simulink model "hopper_6dof"  (R2026b)
settings: Solver=FixedStepAuto  StopTime=tgrid(end)  FixedStep=1e-3  RelTol=1e-5
undefined symbols (not defined in the file): cg_init, controller_start_time, fdir_params, fsw_latency, fsw_period, g, IN, K1flat, K1flat_lo, K2grid, Klqi, nav_dt, nav_g, nav_init, nav_Qc, nav_reset, OUT, p, sensor_params, Target_Trajectory, tgrid, u_hold_command, unom, VEH
libraries: fl_lib x43, nesl_utility x31, SimscapeFluids_lib x13, slpidlib x3, simulink_extras x2, commrandsrc3 x1, dspsrcs4 x1, matrix_library x1, aerolibutil x1
(part 4 of 6)

== system hopper_6dof/Mass_Propulsion/Propulsion/Propulsion_Fluid_Network/Fluid_Network/FBB ==
  Acuation Delay : TransportDelay  DelayTime=0.075  InitialOutput=1  BufferSize=28672
  Constant5 : Constant  Value=0
  Constant6 : Constant
  F Orifice : SimscapeFluids_lib/Gas/Valves & Orifices/Orifice (G)  orifice_type=foundation.enum.constant_variable.constant  orifice_parameterization=fluids.gas.valves_orifices.enum.OrificeParameterization.Area  opening_characteristic=fluids.gas.valves_orifices.enum.OpeningCharacteristics.Linear  Cv_constant=4  Cv_max=4  L_Cv_TLU=0 : 0.2 : 1  Cv_TLU=[1e-06, .8, 1.6, 2.4, 3.2, 4]  xT_Cv=0.7  Kv_constant=3.6  Kv_max=3.6  L_Kv_TLU=0 : 0.2 : 1  Kv_TLU=[1e-06, .72, 1.44, 2.16, 2.88, 3.6]  xT_Kv=0.7  C_constant=12 l/(bar*s)  B_crit_constant=0.3  C_max=12 l/(bar*s)  B_crit_linear=0.3  L_C_TLU=0 : 0.2 : 1  C_TLU=[1e-05, 2.4, 4.8, 7.2, 9.6, 12] l/(bar*s)  B_crit_TLU=0.3 * ones(1, 6)  m=0.5  T_ref_C=293.15 K  rho_ref_C=1.185 kg/m^3  orifice_area_constant=0.025477 in^2  orifice_area_max=1e-4 m^2  L_orifice_area_TLU=0 : 0.2 : 1  orifice_area_TLU=[1e-10, 2e-05, 4e-05, 6e-05, 8e-05, .0001] m^2  Cd=1  leakage_fraction=1e-6  smoothing_factor=0.01  B_lam=0.999  area=0.01 m^2
  FBang : SimscapeFluids_lib/Gas/Valves & Orifices/Flow Control Valves/Poppet Valve (G)  valve_seat_geometry=fluids.gas.valves_orifices.flow_control_valves.enum.ValveSeatGeometry.Sharp  cone_angle=120 deg  diam_ball=0.7 in  diam_orifice=0.05351 in  valve_parameterization=fluids.gas.valves_orifices.flow_control_valves.enum.OrificeParameterization.Geometry  Cd=1  Cv_max=4  xT_Cv=0.7  Kv_max=3.6  xT_Kv=0.7  C_max=12 l/(bar*s)  B_crit_linear=0.3  m=0.5  T_ref_C=293.15 K  rho_ref_C=1.185 kg/m^3  leakage_fraction=10^-9  smoothing_factor=0.01  B_lam=0.999  area=0.78 in^2  x0=0
  FTPT : Scope  Commented=on
      settings: ActiveDisplayYMinimum=469.21439817536259  ActiveDisplayYMaximum=560.55853932482523  DataLoggingVariableName=ScopeData5
  Mass & Energy Flow Rate Sensor (G)1 : fl_lib/Gas/Sensors/Flow Rate Sensor (G)  mass_flow_measure=true  volumetric_flow_measure=false  volumetric_flow_conditions=foundation.enum.volumetric_flow_conditions.actual  p_std=0.101325 MPa  T_std=20 degC  energy_flow_measure=true
  PS-Simulink Converter8 : nesl_utility/PS-Simulink Converter  PhysicalDomain=network_engine_domain  SubClassName=ps_output  LeftPortType=input  RightPortType=output  PseudoPeriodic=off  Frequencies=[]  VectorFormat=inherit  Unit=inherit  AffineConversion=off
  Pipe (G) : fl_lib/Gas/Elements/Pipe (G)  length=0.5 ft  area=0.049 in^2  Dh=0.25 in  length_add=0.1 m  roughness=0.0015 mm  Re_lam=2000  Re_tur=4000  shape_factor=64  Nu_lam=3.66  dynamic_compressibility=true  inertia=false  p_init=4500 psi  p_init_priority=foundation.enum.Priority.High  T_init=293.15 K  T_init_priority=foundation.enum.Priority.High  mdot_init=0 kg/s  mdot_init_priority=foundation.enum.Priority.High  p_nominal=0.101325 MPa  T_nominal=293.15 K
  Pressurant Mass Flow Rate FSide : Scope  Commented=on
      settings: ActiveDisplayYMinimum=-1  ActiveDisplayYMaximum=1  DataLoggingVariableName=ScopeData15
  Rate Limiter1 : RateLimiter  RisingSlewLimit=100  FallingSlewLimit=-100  SampleTimeMode=inherited
  Simulink-PS Converter4 : nesl_utility/Simulink-PS Converter  PhysicalDomain=network_engine_domain  SubClassName=ps_input  LeftPortType=input  RightPortType=output  PseudoPeriodic=off  Frequencies=[]  NoiseDistribution=none  NoiseParameters=[]  Unit=1  AffineConversion=off  FilteringAndDerivatives=filter  SimscapeFilterOrder=1  InputFilterTimeConstant=0.001  UdotUserProvided=0
  Subsystem Reference : Subsystem  ReferencedSubsystem=PT  max_press=5000  lower_val=4  upper_val=20
  Switch1 : Switch  Criteria=u2 > Threshold  Threshold=500  SaturateOnIntegerOverflow=off  InputSameDT=off
  Valve State3 : Scope  Commented=on
      settings: ActiveDisplayYMinimum=-1  ActiveDisplayYMaximum=1  DataLoggingVariableName=ScopeData16
  Conn2 : PMIOPort  Side=Right
  Conn3 : PMIOPort  Port=2  Side=Left
  wires:
  Acuation Delay/1 -> Rate Limiter1/1
  Rate Limiter1/1 -> Valve State3/1, Simulink-PS Converter4/1
  Constant5/1 -> Switch1/1
  PS-Simulink Converter8/1 -> Pressurant Mass Flow Rate FSide/1
  Switch1/1 -> Acuation Delay/1
  Constant6/1 -> Switch1/3
  Subsystem Reference/1 -> FTPT/1, Switch1/2
  connections:
  Pipe (G)/RConn1 -- FBang/LConn1
  Conn3/RConn1 -- Pipe (G)/LConn1
  Mass & Energy Flow Rate Sensor (G)1/RConn1 -- Conn2/RConn1
  F Orifice/LConn1 -- FBang/RConn1
  FBang/LConn2 -- Simulink-PS Converter4/RConn1
  Subsystem Reference/LConn1 -- Mass & Energy Flow Rate Sensor (G)1/LConn1 -- F Orifice/RConn1
  PS-Simulink Converter8/LConn1 -- Mass & Energy Flow Rate Sensor (G)1/RConn2

== system hopper_6dof/Mass_Propulsion/Propulsion/Propulsion_Fluid_Network/Fluid_Network/Fuel Tank ==
  Fuel CdA : SimscapeFluids_lib/Thermal Liquid/Valves & Orifices/Orifice (TL)  Commented=on  orifice_type=foundation.enum.constant_variable.constant  constant_orifice_spec=fluids.thermal_liquid.valves.enum.ConstantOrificeSpec.Area  variable_orifice_spec=fluids.thermal_liquid.valves.enum.orifice_spec.linear  orifice_area_constant=100 mm^2  p_diff_TLU_constant=[-4, -3, -2, -1, -.5, 0, .5, 1, 2, 3, 4] MPa  vol_flow_TLU_constant=[-2.44, -2.12, -1.68, -1.22, -.84, 0, .85, 1.21, 1.7, 2.09, 2.41] .* 1e-3 m^3/s  mdot_TLU_constant=[-2.44, -2.12, -1.68, -1.22, -.84, 0, .85, 1.21, 1.7, 2.09, 2.41] kg/s  S_min=0 m  del_S=5e-3 m  open_orientation=fluids.thermal_liquid.valves.enum.orifice_orientation.positive  area_max=1e-4 m^2  area_leak=1e-10 m^2  S_TLU=[0, .002, .004, .007, .017] m  orifice_area_TLU=[1e-09, 2.0352e-07, 4.0736e-05, .00011438, .00034356] m^2  Cd=1  Re_c=150  smoothing_factor=0.01  pressure_recovery=simscape.enum.onoff.off  S_flow_TLU=[0, .002, .004, .007, .017] m  p_diff_TLU=[.3, .5, .7] MPa  vol_flow_TLU=1e-3 * [1.7e-05, 2e-05, 2.6e-05; .0035, .0045, .0053; .7, .9, 1.06; 1.96, 2.5, 3; 6, 7.7, 9.13] m^3/s  mdot_TLU=[1.7e-05, 2e-05, 2.6e-05; .0035, .0045, .0053; .7, .9, 1.06; 1.96, 2.5, 3; 6, 7.7, 9.13] kg/s  T_ref_in=293.15 K  p_ref_in=0.101325 MPa  area=0.01 m^2
  Fuel CdA1 : SimscapeFluids_lib/Thermal Liquid/Valves & Orifices/Orifice (TL)  orifice_type=foundation.enum.constant_variable.constant  constant_orifice_spec=fluids.thermal_liquid.valves.enum.ConstantOrificeSpec.Area  variable_orifice_spec=fluids.thermal_liquid.valves.enum.orifice_spec.linear  orifice_area_constant=100 mm^2  p_diff_TLU_constant=[-4, -3, -2, -1, -.5, 0, .5, 1, 2, 3, 4] MPa  vol_flow_TLU_constant=[-2.44, -2.12, -1.68, -1.22, -.84, 0, .85, 1.21, 1.7, 2.09, 2.41] .* 1e-3 m^3/s  mdot_TLU_constant=[-2.44, -2.12, -1.68, -1.22, -.84, 0, .85, 1.21, 1.7, 2.09, 2.41] kg/s  S_min=0 m  del_S=5e-3 m  open_orientation=fluids.thermal_liquid.valves.enum.orifice_orientation.positive  area_max=1e-4 m^2  area_leak=1e-10 m^2  S_TLU=[0, .002, .004, .007, .017] m  orifice_area_TLU=[1e-09, 2.0352e-07, 4.0736e-05, .00011438, .00034356] m^2  Cd=1  Re_c=150  smoothing_factor=0.01  pressure_recovery=simscape.enum.onoff.off  S_flow_TLU=[0, .002, .004, .007, .017] m  p_diff_TLU=[.3, .5, .7] MPa  vol_flow_TLU=1e-3 * [1.7e-05, 2e-05, 2.6e-05; .0035, .0045, .0053; .7, .9, 1.06; 1.96, 2.5, 3; 6, 7.7, 9.13] m^3/s  mdot_TLU=[1.7e-05, 2e-05, 2.6e-05; .0035, .0045, .0053; .7, .9, 1.06; 1.96, 2.5, 3; 6, 7.7, 9.13] kg/s  T_ref_in=293.15 K  p_ref_in=0.101325 MPa  area=0.01 m^2
  Fuel Liquid Level : Scope  Commented=on
      settings: ActiveDisplayYMinimum=-0.022349805039863307  ActiveDisplayYMaximum=0.600478334821636  DataLoggingVariableName=ScopeData6
  Fuel Mass Flow Rate : Scope  Commented=on
      settings: ActiveDisplayYMinimum=-0.023909818576535891  ActiveDisplayYMaximum=0.21591293735607325  DataLoggingVariableName=ScopeData7
  Fuel Mass Rate : Scope  Commented=on
      settings: ActiveDisplayYMinimum=-7.0412281631605644  ActiveDisplayYMaximum=46.559064275310185  DataLoggingVariableName=ScopeData18
  Fuel Tank (Jet A) : SimscapeFluids_lib/Thermal Liquid/Tanks & Accumulators/Tank (G-TL)  num_inlet=1  volume_total=30 l  volume_spec=fluids.thermal_liquid.tanks_accumulators.enum.TankVolumeSpec.Constant  tank_area=0.35 ft^2  level_TLU=[0, 3, 5] m  volume_TLU=[0, 4, 6] m^3  inlet_areas_A1B1=[1, 1] in^2  inlet_height_A2=0 m  inlet_area_A2=0.78 in^2  inlet_heights_A2B2=[.1, .1] m  inlet_areas_A2B2=[.01, .01] m^2  inlet_heights_A2B2C2=[.1, .1, .1] m  inlet_areas_A2B2C2=[.01, .01, .01] m^2  inlet_heights_A2B2C2D2=0.1 * ones(1, 4) m  inlet_areas_A2B2C2D2=0.01 * ones(1, 4) m^2  inlet_heights_A2B2C2D2E2=0.1 * ones(1, 5) m  inlet_areas_A2B2C2D2E2=0.01 * ones(1, 5) m^2  inlet_heights_A2B2C2D2E2F2=0.1 * ones(1, 6) m  inlet_areas_A2B2C2D2E2F2=0.01 * ones(1, 6) m^2  capacity_check=0  max_liquid_capacity=55 l  g=9.81 m/s^2  level_specify=off  level_priority=None  level=19 in  level_nominal_specify=off  level_nominal_value=1  level_nominal_unit=m  volume_liquid_specify=off  volume_liquid_priority=None  volume_liquid=15.18 l  volume_liquid_nominal_specify=off  volume_liquid_nominal_value=1  volume_liquid_nominal_unit=m^3  mass_liquid_specify=on  mass_liquid_priority=High  mass_liquid=20 kg  mass_liquid_nominal_specify=off  mass_liquid_nominal_value=1  mass_liquid_nominal_unit=kg  T_liquid_specify=off  T_liquid_priority=High  T_liquid=293.15 K  T_liquid_nominal_specify=off  T_liquid_nominal_value=1  T_liquid_nominal_unit=K  p_gas_specify=on  p_gas_priority=High  p_gas=500 psi  p_gas_nominal_specify=off  p_gas_nominal_value=1  p_gas_nominal_unit=MPa  T_gas_specify=off  T_gas_priority=High  T_gas=293.15 K  T_gas_nominal_specify=off  T_gas_nominal_value=1  T_gas_nominal_unit=K  rho_gas_specify=off  rho_gas_priority=None  rho_gas=1.2 kg/m^3  rho_gas_nominal_specify=off  rho_gas_nominal_value=1  rho_gas_nominal_unit=kg/m^3
  Integrator : Integrator  Commented=on
  Jet A Properties : fl_lib/Thermal Liquid/Utilities/Thermal Liquid Settings (TL)  table_dimensions=1  T_TLU=[273.1600 : 10 : 373.16]' K  p_TLU=[0.01, 0.1, 5 : 5 : 50] MPa  T_atm=293.15 K  p_atm=0.101325 MPa  pT_region_flag=0  T_min=273.16 K  T_max=363.16 K  p_min=0.05 MPa  p_max=50 MPa  T_min_1D=273.16 K  T_max_1D=373.16 K  p_min_1D=0.01 MPa  p_max_1D=50 MPa  pT_validity_TLU=[1, 1, 1, 1, 1, 1, 1, 1, 1, 1, 1, 1; 1, 1, 1, 1, 1, 1, 1, 1, 1, 1, 1, 1; 1, 1, 1, 1, 1, 1, 1, 1, 1, 1, 1, 1; 1, 1, 1, 1, 1, 1, 1, 1, 1, 1, 1, 1; 1, 1, 1, 1, 1, 1, 1, 1, 1, 1, 1, 1; 0, 1, 1, 1, 1, 1, 1, 1, 1, 1, 1, 1; 0, 1, 1, 1, 1, 1, 1, 1, 1, 1, 1, 1; 0, 1, 1, 1, 1, 1, 1, 1, 1, 1, 1, 1; 0, 1, 1, 1, 1, 1, 1, 1, 1, 1, 1, 1; 0, 1, 1, 1, 1, 1, 1, 1, 1, 1, 1, 1; 0, 0, 1, 1, 1, 1, 1, 1, 1, 1, 1, 1]  properties_range_check=simscape.enum.assert.action.error  rho_parameterization_2D=1  rho_parameterization_1D=2  rho_TLU=[999.7973, 999.8431, 1002.3216, 1004.8218, 1007.293, 1009.7358, 1012.1506, 1014.5379, 1016.8979, 1019.2311, 1021.538, 1023.8188; 999.6579, 999.7009, 1002.0303, 1004.382, 1006.7084, 1009.0101, 1011.2874, 1013.5407, 1015.7703, 1017.9766, 1020.1599, 1022.3206; 998.1632, 998.2045, 1000.4375, 1002.6924, 1004.9239, 1007.1324, 1009.3183, 1011.4819, 1013.6236, 1015.7438, 1017.8428, 1019.921; 995.6057, 995.6458, 997.81864, 1000.0128, 1002.1841, 1004.3332, 1006.4603, 1008.566, 1010.6505, 1012.7144, 1014.758, 1016.7815; 992.1724, 992.2119, 994.35133, 996.5113, 998.6484, 1000.7633, 1002.8563, 1004.928, 1006.9788, 1009.009, 1011.0192, 1013.0097; 988.02, 988.0299, 990.15684, 992.3035, 994.4268, 996.5273, 998.6056, 1000.6622, 1002.6976, 1004.7123, 1006.7067, 1008.6813; 983.18, 983.1901, 985.3217, 987.4721, 989.5983, 991.7008, 993.7803, 995.8374, 997.8726, 999.8864, 1001.8795, 1003.8522; 977.75, 977.7583, 979.9094, 982.0783, 984.2216, 986.34, 988.4343, 990.505, 992.5529, 994.5786, 996.5825, 998.5654; 971.77, 971.7836, 973.96734, 976.1678, 978.3409, 980.4876, 982.6087, 984.7049, 986.7768, 988.8254, 990.8511, 992.8545; 965.26, 965.3023, 967.53107, 969.7753, 971.9901, 974.1764, 976.3354, 978.4676, 980.5741, 982.6556, 984.7129, 986.7465; 958.62, 958.6315, 960.627, 962.9267, 965.1944, 967.4314, 969.6387, 971.8173, 973.9681, 976.0921, 978.19, 980.2628] kg/m^3  beta_TLU=[1.9649, 1.9654, 1.9929, 2.0213, 2.0499, 2.0787, 2.1078, 2.1372, 2.1668, 2.1966, 2.2268, 2.2572; 2.0913, 2.0918, 2.1191, 2.1471, 2.1752, 2.2036, 2.2322, 2.261, 2.2899, 2.3191, 2.3485, 2.3781; 2.1786, 2.1791, 2.2067, 2.235, 2.2634, 2.2919, 2.3206, 2.3494, 2.3784, 2.4075, 2.4367, 2.4661; 2.2332, 2.2337, 2.2619, 2.2908, 2.3197, 2.3487, 2.3778, 2.407, 2.4363, 2.4657, 2.4951, 2.5246; 2.26, 2.2605, 2.2895, 2.3191, 2.3487, 2.3784, 2.4081, 2.4378, 2.4675, 2.4973, 2.5272, 2.5571; 2.2638, 2.2638, 2.2936, 2.324, 2.3544, 2.3848, 2.4151, 2.4455, 2.4758, 2.5062, 2.5365, 2.5669; 2.2472, 2.2472, 2.2779, 2.3092, 2.3403, 2.3715, 2.4025, 2.4336, 2.4646, 2.4955, 2.5264, 2.5573; 2.214, 2.214, 2.2455, 2.2776, 2.3096, 2.3415, 2.3733, 2.405, 2.4367, 2.4683, 2.4998, 2.5313; 2.1668, 2.1668, 2.1992, 2.2321, 2.2649, 2.2976, 2.3301, 2.3626, 2.3949, 2.4272, 2.4593, 2.4914; 2.1081, 2.1081, 2.1413, 2.175, 2.2086, 2.2421, 2.2754, 2.3085, 2.3415, 2.3744, 2.4072, 2.4399; 2.0494, 2.0494, 2.0739, 2.1084, 2.1428, 2.177, 2.211, 2.2449, 2.2786, 2.3121, 2.3455, 2.3788] GPa  alpha_TLU=1e-4 * [-.679, -.676, -.49, -.307, -.13, .041, .206, .365, .519, .668, .811, .949; .878, .881, .998, 1.114, 1.227, 1.337, 1.445, 1.549, 1.651, 1.75, 1.846, 1.939; 2.068, 2.069, 2.141, 2.213, 2.283, 2.352, 2.42, 2.486, 2.551, 2.614, 2.676, 2.736; 3.034, 3.035, 3.074, 3.113, 3.152, 3.191, 3.229, 3.267, 3.305, 3.341, 3.377, 3.413; 3.855, 3.856, 3.87, 3.884, 3.899, 3.914, 3.93, 3.946, 3.961, 3.977, 3.993, 4.009; 4.578, 4.578, 4.572, 4.566, 4.562, 4.558, 4.555, 4.552, 4.55, 4.549, 4.548, 4.547; 5.233, 5.233, 5.209, 5.186, 5.165, 5.144, 5.125, 5.107, 5.09, 5.074, 5.059, 5.045; 5.84, 5.84, 5.801, 5.762, 5.725, 5.691, 5.657, 5.625, 5.595, 5.566, 5.538, 5.512; 6.414, 6.414, 6.36, 6.307, 6.256, 6.208, 6.161, 6.117, 6.074, 6.033, 5.994, 5.956; 6.967, 6.967, 6.898, 6.831, 6.766, 6.705, 6.646, 6.589, 6.535, 6.482, 6.432, 6.384; 7.519, 7.519, 7.423, 7.342, 7.264, 7.189, 7.118, 7.049, 6.983, 6.92, 6.859, 6.8] 1/K  rho_TLU_2=[999.7973, 999.8431, 1002.3216, 1004.8218, 1007.293, 1009.7358, 1012.1506, 1014.5379, 1016.8979, 1019.2311, 1021.538, 1023.8188; 999.6579, 999.7009, 1002.0303, 1004.382, 1006.7084, 1009.0101, 1011.2874, 1013.5407, 1015.7703, 1017.9766, 1020.1599, 1022.3206; 998.1632, 998.2045, 1000.4375, 1002.6924, 1004.9239, 1007.1324, 1009.3183, 1011.4819, 1013.6236, 1015.7438, 1017.8428, 1019.921; 995.6057, 995.6458, 997.81864, 1000.0128, 1002.1841, 1004.3332, 1006.4603, 1008.566, 1010.6505, 1012.7144, 1014.758, 1016.7815; 992.1724, 992.2119, 994.35133, 996.5113, 998.6484, 1000.7633, 1002.8563, 1004.928, 1006.9788, 1009.009, 1011.0192, 1013.0097; 988.02, 988.0299, 990.15684, 992.3035, 994.4268, 996.5273, 998.6056, 1000.6622, 1002.6976, 1004.7123, 1006.7067, 1008.6813; 983.18, 983.1901, 985.3217, 987.4721, 989.5983, 991.7008, 993.7803, 995.8374, 997.8726, 999.8864, 1001.8795, 1003.8522; 977.75, 977.7583, 979.9094, 982.0783, 984.2216, 986.34, 988.4343, 990.505, 992.5529, 994.5786, 996.5825, 998.5654; 971.77, 971.7836, 973.96734, 976.1678, 978.3409, 980.4876, 982.6087, 984.7049, 986.7768, 988.8254, 990.8511, 992.8545; 965.26, 965.3023, 967.53107, 969.7753, 971.9901, 974.1764, 976.3354, 978.4676, 980.5741, 982.6556, 984.7129, 986.7465; 958.62, 958.6315, 960.627, 962.9267, 965.1944, 967.4314, 969.6387, 971.8173, 973.9681, 976.0921, 978.19, 980.2628] kg/m^3  rho_ref_3=998.21 kg/m^3  T_ref_3=293.16 K  p_ref_3=0.101325 MPa  beta_const_3=2.1791 GPa  alpha_const_3=2.0691e-4 1/K  rho_TLU_4=[999.84; 999.7; 998.2; 995.65; 992.21; 988.03; 983.19; 977.76; 971.78; 965.3; 958.8] kg/m^3  beta_const_4=2.1791 GPa  p_ref_4=0.101325 MPa  rho_ref_5=FuelProps.rho_ref kg/m^3  T_ref_5=FuelProps.T_ref K  p_ref_5=FuelProps.p_ref MPa  beta_const_5=FuelProps.beta Pa  alpha_const_5=FuelProps.alpha 1/K  u_parameterization_2D=1  u_parameterization_1D=2  u_TLU=[.0002, .0018, .086, .1588, .219, .267, .3034, .3288, .3436, .3483, .3435, .3294; 42.062, 42.06, 41.935, 41.804, 41.668, 41.527, 41.382, 41.233, 41.081, 40.924, 40.763, 40.599; 83.953, 83.948, 83.651, 83.349, 83.049, 82.749, 82.451, 82.153, 81.856, 81.56, 81.265, 80.971; 125.77, 125.76, 125.31, 124.86, 124.41, 123.97, 123.53, 123.1, 122.68, 122.25, 121.84, 121.42; 167.57, 167.56, 166.96, 166.37, 165.79, 165.21, 164.65, 164.09, 163.54, 163, 162.46, 161.94; 209.36, 209.36, 208.63, 207.9, 207.19, 206.48, 205.79, 205.11, 204.45, 203.79, 203.14, 202.5; 251.19, 251.19, 250.33, 249.47, 248.62, 247.79, 246.98, 246.18, 245.39, 244.62, 243.86, 243.12; 293.06, 293.06, 292.07, 291.07, 290.1, 289.14, 288.2, 287.28, 286.38, 285.49, 284.62, 283.77; 334.99, 334.99, 333.86, 332.73, 331.63, 330.54, 329.48, 328.44, 327.41, 326.41, 325.43, 324.46; 377, 377, 375.73, 374.46, 373.22, 372, 370.81, 369.64, 368.5, 367.38, 366.27, 365.19; 419.01, 419.01, 417.69, 416.27, 414.89, 413.54, 412.21, 410.91, 409.64, 408.4, 407.17, 405.98] kJ/kg  cp_TLU=[4.2199, 4.2194, 4.1957, 4.1726, 4.1508, 4.13, 4.1103, 4.0916, 4.0738, 4.0569, 4.0408, 4.0254; 4.1955, 4.1951, 4.1769, 4.1592, 4.1422, 4.1259, 4.1103, 4.0954, 4.0812, 4.0676, 4.0545, 4.0421; 4.1843, 4.184, 4.169, 4.1543, 4.1401, 4.1264, 4.1133, 4.1007, 4.0885, 4.0768, 4.0656, 4.0548; 4.1801, 4.1798, 4.1667, 4.1538, 4.1413, 4.1293, 4.1177, 4.1064, 4.0956, 4.0851, 4.075, 4.0653; 4.1796, 4.1794, 4.1675, 4.1558, 4.1444, 4.1334, 4.1227, 4.1123, 4.1023, 4.0926, 4.0832, 4.0741; 4.1813, 4.1813, 4.1702, 4.1592, 4.1484, 4.138, 4.1279, 4.1181, 4.1086, 4.0993, 4.0903, 4.0816; 4.185, 4.185, 4.1742, 4.1636, 4.1532, 4.1432, 4.1334, 4.1239, 4.1146, 4.1056, 4.0969, 4.0884; 4.1901, 4.1901, 4.1795, 4.169, 4.1588, 4.1489, 4.1393, 4.1299, 4.1207, 4.1118, 4.1032, 4.0947; 4.1968, 4.1968, 4.1862, 4.1757, 4.1655, 4.1555, 4.1458, 4.1364, 4.1273, 4.1183, 4.1096, 4.1012; 4.2052, 4.2052, 4.1944, 4.1837, 4.1733, 4.1632, 4.1534, 4.1438, 4.1345, 4.1255, 4.1166, 4.108; 4.2136, 4.2136, 4.2045, 4.1935, 4.1828, 4.1724, 4.1623, 4.1524, 4.1429, 4.1335, 4.1245, 4.1157] kJ/kg/K  u_TLU_2=[.0002, .0018, .086, .1588, .219, .267, .3034, .3288, .3436, .3483, .3435, .3294; 42.062, 42.06, 41.935, 41.804, 41.668, 41.527, 41.382, 41.233, 41.081, 40.924, 40.763, 40.599; 83.953, 83.948, 83.651, 83.349, 83.049, 82.749, 82.451, 82.153, 81.856, 81.56, 81.265, 80.971; 125.77, 125.76, 125.31, 124.86, 124.41, 123.97, 123.53, 123.1, 122.68, 122.25, 121.84, 121.42; 167.57, 167.56, 166.96, 166.37, 165.79, 165.21, 164.65, 164.09, 163.54, 163, 162.46, 161.94; 209.36, 209.36, 208.63, 207.9, 207.19, 206.48, 205.79, 205.11, 204.45, 203.79, 203.14, 202.5; 251.19, 251.19, 250.33, 249.47, 248.62, 247.79, 246.98, 246.18, 245.39, 244.62, 243.86, 243.12; 293.06, 293.06, 292.07, 291.07, 290.1, 289.14, 288.2, 287.28, 286.38, 285.49, 284.62, 283.77; 334.99, 334.99, 333.86, 332.73, 331.63, 330.54, 329.48, 328.44, 327.41, 326.41, 325.43, 324.46; 377, 377, 375.73, 374.46, 373.22, 372, 370.81, 369.64, 368.5, 367.38, 366.27, 365.19; 419.01, 419.01, 417.69, 416.27, 414.89, 413.54, 412.21, 410.91, 409.64, 408.4, 407.17, 405.98] kJ/kg  cp_TLU_3=[4.2199, 4.2194, 4.1957, 4.1726, 4.1508, 4.13, 4.1103, 4.0916, 4.0738, 4.0569, 4.0408, 4.0254; 4.1955, 4.1951, 4.1769, 4.1592, 4.1422, 4.1259, 4.1103, 4.0954, 4.0812, 4.0676, 4.0545, 4.0421; 4.1843, 4.184, 4.169, 4.1543, 4.1401, 4.1264, 4.1133, 4.1007, 4.0885, 4.0768, 4.0656, 4.0548; 4.1801, 4.1798, 4.1667, 4.1538, 4.1413, 4.1293, 4.1177, 4.1064, 4.0956, 4.0851, 4.075, 4.0653; 4.1796, 4.1794, 4.1675, 4.1558, 4.1444, 4.1334, 4.1227, 4.1123, 4.1023, 4.0926, 4.0832, 4.0741; 4.1813, 4.1813, 4.1702, 4.1592, 4.1484, 4.138, 4.1279, 4.1181, 4.1086, 4.0993, 4.0903, 4.0816; 4.185, 4.185, 4.1742, 4.1636, 4.1532, 4.1432, 4.1334, 4.1239, 4.1146, 4.1056, 4.0969, 4.0884; 4.1901, 4.1901, 4.1795, 4.169, 4.1588, 4.1489, 4.1393, 4.1299, 4.1207, 4.1118, 4.1032, 4.0947; 4.1968, 4.1968, 4.1862, 4.1757, 4.1655, 4.1555, 4.1458, 4.1364, 4.1273, 4.1183, 4.1096, 4.1012; 4.2052, 4.2052, 4.1944, 4.1837, 4.1733, 4.1632, 4.1534, 4.1438, 4.1345, 4.1255, 4.1166, 4.108; 4.2136, 4.2136, 4.2045, 4.1935, 4.1828, 4.1724, 4.1623, 4.1524, 4.1429, 4.1335, 4.1245, 4.1157] kJ/kg/K  u_TLU_4=[.0018; 42.06; 83.948; 125.76; 167.56; 209.36; 251.19; 293.06; 334.99; 377; 418.01] kJ/kg  cp_TLU_5=FuelProps.cp_TLU kJ/kg/K  nu_TLU=[1.7917, 1.7914, 1.7763, 1.7615, 1.7473, 1.7338, 1.7208, 1.7085, 1.6967, 1.6854, 1.6747, 1.6645; 1.3061, 1.3059, 1.2986, 1.2914, 1.2845, 1.2779, 1.2716, 1.2656, 1.2598, 1.2543, 1.2491, 1.2441; 1.0032, 1.0032, .9995, .9959, .9924, .9891, .9859, .9829, .9801, .9774, .9748, .9724; .8006, .8005, .7987, .797, .7953, .7937, .7922, .7908, .7894, .7881, .787, .7859; .6577, .6577, .657, .6562, .6555, .6548, .6543, .6537, .6532, .6528, .6523, .652; .553, .553, .5529, .5527, .5526, .5525, .5524, .5524, .5524, .5524, .5524, .5525; .4739, .4739, .4741, .4743, .4745, .4747, .475, .4753, .4755, .4758, .4762, .4765; .4127, .4127, .4131, .4135, .4139, .4143, .4148, .4152, .4157, .4162, .4167, .4172; .3643, .3643, .3648, .3654, .3659, .3665, .367, .3676, .3682, .3688, .3694, .37; .3254, .3254, .3261, .3267, .3273, .328, .3286, .3293, .3299, .3306, .3312, .3319; .2866, .2866, .2945, .2952, .2959, .2965, .2972, .2979, .2986, .2993, .3, .3007] mm^2/s  nu_TLU_2=FuelProps.nu_TLU cSt  k_TLU=[561.04, 561.09, 563.8, 566.56, 569.32, 572.08, 574.82, 577.54, 580.24, 582.92, 585.57, 588.18; 580.02, 580.07, 582.45, 584.88, 587.32, 589.75, 592.18, 594.61, 597.02, 599.42, 601.8, 604.16; 598.44, 598.48, 600.73, 603.03, 605.33, 607.64, 609.94, 612.24, 614.54, 616.82, 619.1, 621.36; 615.48, 615.52, 617.73, 620, 622.26, 624.54, 626.81, 629.07, 631.34, 633.6, 635.85, 638.09; 630.6, 630.64, 632.87, 635.15, 637.44, 639.72, 642.01, 644.29, 646.57, 648.84, 651.11, 653.36; 643.61, 643.61, 645.88, 648.21, 650.53, 652.86, 655.18, 657.51, 659.82, 662.14, 664.44, 666.74; 654.39, 654.39, 656.73, 659.12, 661.5, 663.89, 666.27, 668.65, 671.02, 673.38, 675.74, 678.09; 663.13, 663.13, 665.54, 668, 670.46, 672.91, 675.36, 677.8, 680.24, 682.67, 685.09, 687.5; 670.02, 670.02, 672.51, 675.05, 677.59, 680.12, 682.64, 685.16, 687.67, 690.17, 692.66, 695.14; 675.27, 675.27, 677.85, 680.48, 683.11, 685.73, 688.34, 690.94, 693.53, 696.11, 698.68, 701.24; 680.52, 680.52, 681.77, 684.5, 687.22, 689.94, 692.64, 695.34, 698.02, 700.69, 703.35, 706] mW/m/K  k_TLU_2=FuelProps.k_TLU W/(m*K)  air_fraction=0  R_air=0.287 kJ/(K*kg)  air_dissolution_model=false  p_crit=3 MPa
  Mass & Energy Flow Rate Sensor (TL) : fl_lib/Thermal Liquid/Sensors/Flow Rate Sensor (TL)  Commented=on  mass_flow_measure=true  volumetric_flow_measure=false  energy_flow_measure=true
  PS-Simulink Converter : nesl_utility/PS-Simulink Converter  Commented=on  PhysicalDomain=network_engine_domain  SubClassName=ps_output  LeftPortType=input  RightPortType=output  PseudoPeriodic=off  Frequencies=[]  VectorFormat=inherit  Unit=inherit  AffineConversion=off
  PS-Simulink Converter5 : nesl_utility/PS-Simulink Converter  Commented=on  PhysicalDomain=network_engine_domain  SubClassName=ps_output  LeftPortType=input  RightPortType=output  PseudoPeriodic=off  Frequencies=[]  VectorFormat=inherit  Unit=inherit  AffineConversion=off
  Pipe (TL) : fl_lib/Thermal Liquid/Elements/Pipe (TL)  length=0.5 ft  area=0.049 in^2  Dh=0.025 in  length_add=1 m  roughness=15e-6 m  Re_lam=2000  Re_tur=4000  shape_factor=64  Nu_lam=3.66  dynamic_compressibility=true  inertia=false  p0=500 psi  T0=293.15 K  mdot0=0 kg/s  p_nominal=0.101325 MPa  T_nominal=293.15 K
  Solver Configuration : nesl_utility/Solver Configuration  PhysicalDomain=network_engine_domain  SubClassName=solver  LeftPortType=input  RightPortType=generic  Tones=[]  Harmonics=[]  SimulateNoise=off  Profile=off  UseLocalSampling=off  EnableSwitchedLinearOptims=on  FrequencyDomain=off  UseCCode=off  RelTol=0.001  AbsTol=0.001  MinStep=1e-09  ToWorkspace=off  RevertToSquareIcSolve=off  NumHomotopyIterations=100  PhasorMode=off  PhasorModeNumHarmonics=1  ConsistencySolver=NEWTON_XTOL_AFTER_FTOL  CanonicalOrdering=UNORDERED  OptimizeIntermediates=UNOPTIMIZED  MulticoreSolverChoice=BACKWARD_EULER  IndexReductionMethod=DerivativeReplacement  DoDC=off  ResidualTolerance=1e-09  ConsistencyTolSource=GLOBAL  ConsistencyAbsTol=0.001  ConsistencyRelTol=0.001  ConsistencyTolFactor=0.0001  UseLocalSolver=on  LocalSolverChoice=NE_BACKWARD_EULER_ADVANCER  ResolveIndetEquations=on  FunctionEvalNumThread=1  LocalSolverSampleTime=0.001  DoFixedCost=off  MaxNonlinIter=3  MaxModeIter=2  ComputeImpulses=off  ImpulseIterations=2  LinearAlgebra=auto  LinearAlgebraNumThread=0  EquationFormulation=NE_TIME_EF  DelaysMemoryBudget=1024  AutomaticFiltering=on  FilteringTimeConstant=0.001  PartitionStorageMethod=AS_NEEDED  PartitionMemoryBudget=1024  PartitionMethod=BALANCED  MultibodyUseLocalSolver=off  MultibodyLocalSolverChoice=ODE1  MultibodyLocalSolverSampleTime=0.001
  Sum : Sum  Commented=on  Inputs=|-+
  starting mass : Constant  Commented=on  Value=9.7
  Conn2 : PMIOPort  Side=Left
  Conn6 : PMIOPort  Port=2  Side=Right
  wires:
  Sum/1 -> Fuel Mass Rate/1
  Integrator/1 -> Sum/1
  starting mass/1 -> Sum/2
  PS-Simulink Converter5/1 -> Fuel Mass Flow Rate/1, Integrator/1
  PS-Simulink Converter/1 -> Fuel Liquid Level/1
  connections:
  Fuel CdA1/RConn1 -- Conn6/RConn1
  Fuel Tank (Jet A)/LConn3 -- Solver Configuration/RConn1 -- Fuel CdA1/LConn1 -- Jet A Properties/RConn1
  Mass & Energy Flow Rate Sensor (TL)/LConn1 -- Fuel CdA/RConn1
  Conn2/RConn1 -- Fuel Tank (Jet A)/LConn1
  Fuel Tank (Jet A)/LConn5 -- PS-Simulink Converter/LConn1
  PS-Simulink Converter5/LConn1 -- Mass & Energy Flow Rate Sensor (TL)/RConn2

== system hopper_6dof/Mass_Propulsion/Propulsion/Propulsion_Fluid_Network/Fluid_Network/Fuel Tank PT + Initial Condition ==
  Initial FT Pressure : InitialCondition  Value=500
  PS-Simulink Converter8 : nesl_utility/PS-Simulink Converter  PhysicalDomain=network_engine_domain  SubClassName=ps_output  LeftPortType=input  RightPortType=output  PseudoPeriodic=off  Frequencies=[]  VectorFormat=inherit  Unit=inherit  AffineConversion=off
  Pa to psi1 : Gain  Gain=0.000145038
  Pressure & Temperature Sensor (TL)2 : fl_lib/Thermal Liquid/Sensors/Pressure & Temperature Sensor (TL)  reference=foundation.enum.MeasurementReference.absolute  pressure=true  pressure_spec=foundation.enum.PressureMeasementSpec.Gauge  temperature=false
  Conn1 : PMIOPort  Side=Left
  Pup : Outport
  wires:
  Initial FT Pressure/1 -> Pup/1
  Pa to psi1/1 -> Initial FT Pressure/1
  PS-Simulink Converter8/1 -> Pa to psi1/1
  connections:
  Pressure & Temperature Sensor (TL)2/LConn1 -- Conn1/RConn1
  Pressure & Temperature Sensor (TL)2/RConn1 -- PS-Simulink Converter8/LConn1

== system hopper_6dof/Mass_Propulsion/Propulsion/Propulsion_Fluid_Network/Fluid_Network/Injector1 ==
  P_down_fuel : Inport
  rho_fuel : Inport  Port=2
  mdot_fuel : Inport  Port=3
  CdA : Inport  Port=4
  Fuel Injector Calculations : MATLAB Function  TreatAsAtomicUnit=on
  Gain3 : Gain  Gain=0.00014504
  Scope : Scope
      settings: ActiveDisplayYMinimum=-12.688196274763053  ActiveDisplayYMaximum=114.19378727350779  DataLoggingVariableName=ScopeData45
  Scope1 : Scope
      settings: ActiveDisplayYMinimum=266586.73316801467  ActiveDisplayYMaximum=767647.88581813406  DataLoggingVariableName=ScopeData47
  fuel stiffness : Outport
  fuel_P_up : Outport  Port=2
  wires:
  Gain3/1 -> Scope/1
  Fuel Injector Calculations/3(dP_inj) -> Gain3/1
  mdot_fuel/1 -> Fuel Injector Calculations/3(mdot)
  CdA/1 -> Fuel Injector Calculations/4(CdA)
  Fuel Injector Calculations/1(stiffness) -> fuel stiffness/1
  Fuel Injector Calculations/2(P_up) -> fuel_P_up/1
  P_down_fuel/1 -> Fuel Injector Calculations/1(P_down), Scope1/1
  rho_fuel/1 -> Fuel Injector Calculations/2(rho)

== system hopper_6dof/Mass_Propulsion/Propulsion/Propulsion_Fluid_Network/Fluid_Network/Injector2 ==
  CdA : Inport
  P_down_ox : Inport  Port=2
  rho_ox : Inport  Port=3
  mdot_ox : Inport  Port=4
  Gain3 : Gain  Gain=0.00014504
  Ox Injector Calculations : MATLAB Function  TreatAsAtomicUnit=on
  Scope : Scope
      settings: ActiveDisplayYMinimum=-1  ActiveDisplayYMaximum=1  DataLoggingVariableName=ScopeData46
  ox stiffness : Outport
  ox_P_up : Outport  Port=2
  wires:
  Gain3/1 -> Scope/1
  Ox Injector Calculations/3(dP_inj) -> Gain3/1
  mdot_ox/1 -> Ox Injector Calculations/3(mdot)
  Ox Injector Calculations/1(stiffness) -> ox stiffness/1
  CdA/1 -> Ox Injector Calculations/4(CdA)
  rho_ox/1 -> Ox Injector Calculations/2(rho)
  P_down_ox/1 -> Ox Injector Calculations/1(P_down)
  Ox Injector Calculations/2(P_up) -> ox_P_up/1

== system hopper_6dof/Mass_Propulsion/Propulsion/Propulsion_Fluid_Network/Fluid_Network/LBB ==
  Acuation Delay2 : TransportDelay  DelayTime=0.01  InitialOutput=1
  Backlash : Backlash
  Constant1 : Constant  Value=0
  Constant2 : Constant
  O Orifice : SimscapeFluids_lib/Gas/Valves & Orifices/Orifice (G)  orifice_type=foundation.enum.constant_variable.constant  orifice_parameterization=fluids.gas.valves_orifices.enum.OrificeParameterization.Area  opening_characteristic=fluids.gas.valves_orifices.enum.OpeningCharacteristics.Linear  Cv_constant=4  Cv_max=4  L_Cv_TLU=0 : 0.2 : 1  Cv_TLU=[1e-06, .8, 1.6, 2.4, 3.2, 4]  xT_Cv=0.7  Kv_constant=3.6  Kv_max=3.6  L_Kv_TLU=0 : 0.2 : 1  Kv_TLU=[1e-06, .72, 1.44, 2.16, 2.88, 3.6]  xT_Kv=0.7  C_constant=12 l/(bar*s)  B_crit_constant=0.3  C_max=12 l/(bar*s)  B_crit_linear=0.3  L_C_TLU=0 : 0.2 : 1  C_TLU=[1e-05, 2.4, 4.8, 7.2, 9.6, 12] l/(bar*s)  B_crit_TLU=0.3 * ones(1, 6)  m=0.5  T_ref_C=293.15 K  rho_ref_C=1.185 kg/m^3  orifice_area_constant=0.0272 in^2  orifice_area_max=1e-4 m^2  L_orifice_area_TLU=0 : 0.2 : 1  orifice_area_TLU=[1e-10, 2e-05, 4e-05, 6e-05, 8e-05, .0001] m^2  Cd=1  leakage_fraction=1e-6  smoothing_factor=0.01  B_lam=0.999  area=0.01 m^2
  OBang : SimscapeFluids_lib/Gas/Valves & Orifices/Flow Control Valves/Poppet Valve (G)  valve_seat_geometry=fluids.gas.valves_orifices.flow_control_valves.enum.ValveSeatGeometry.Sharp  cone_angle=120 deg  diam_ball=0.1 in  diam_orifice=0.07568 in  valve_parameterization=fluids.gas.valves_orifices.flow_control_valves.enum.OrificeParameterization.Geometry  Cd=1  Cv_max=4  xT_Cv=0.7  Kv_max=3.6  xT_Kv=0.7  C_max=12 l/(bar*s)  B_crit_linear=0.3  m=0.5  T_ref_C=293.15 K  rho_ref_C=1.185 kg/m^3  leakage_fraction=10^-9  smoothing_factor=0.01  B_lam=0.999  area=0.78 in^2  x0=0
  OTPT : Scope  Commented=on
      settings: ActiveDisplayYMinimum=481.09324150740861  ActiveDisplayYMaximum=526.62934859347286  DataLoggingVariableName=ScopeData13
  Pipe (G) : fl_lib/Gas/Elements/Pipe (G)  length=0.5 ft  area=0.049 in^2  Dh=0.25 in  length_add=0.1 m  roughness=0.0015 mm  Re_lam=2000  Re_tur=4000  shape_factor=64  Nu_lam=3.66  dynamic_compressibility=true  inertia=false  p_init=4500 psi  p_init_priority=foundation.enum.Priority.High  T_init=293.15 K  T_init_priority=foundation.enum.Priority.High  mdot_init=0 kg/s  mdot_init_priority=foundation.enum.Priority.High  p_nominal=0.101325 MPa  T_nominal=293.15 K
  Rate Limiter3 : RateLimiter  RisingSlewLimit=100  FallingSlewLimit=-100  SampleTimeMode=inherited
  Simulink-PS Converter2 : nesl_utility/Simulink-PS Converter  PhysicalDomain=network_engine_domain  SubClassName=ps_input  LeftPortType=input  RightPortType=output  PseudoPeriodic=off  Frequencies=[]  NoiseDistribution=none  NoiseParameters=[]  Unit=1  AffineConversion=off  FilteringAndDerivatives=filter  SimscapeFilterOrder=1  InputFilterTimeConstant=0.001  UdotUserProvided=0
  Subsystem Reference2 : Subsystem  ReferencedSubsystem=PT  max_press=5000  lower_val=4  upper_val=20
  Switch3 : Switch  Criteria=u2 > Threshold  Threshold=500  SaturateOnIntegerOverflow=off  InputSameDT=off
  Valve State1 : Scope  Commented=on
      settings: ActiveDisplayYMinimum=0.055008171460110944  ActiveDisplayYMaximum=1.034415879545685  DataLoggingVariableName=ScopeData17
  Conn1 : PMIOPort  Side=Left
  Input : PMIOPort  Port=2  Side=Right
  wires:
  Rate Limiter3/1 -> Simulink-PS Converter2/1, Valve State1/1
  Switch3/1 -> Acuation Delay2/1
  Constant2/1 -> Switch3/3
  Acuation Delay2/1 -> Rate Limiter3/1
  Constant1/1 -> Switch3/1
  Subsystem Reference2/1 -> OTPT/1, Switch3/2
  connections:
  Pipe (G)/RConn1 -- OBang/LConn1
  Conn1/RConn1 -- Pipe (G)/LConn1
  OBang/RConn1 -- O Orifice/LConn1
  O Orifice/RConn1 -- Input/RConn1 -- Subsystem Reference2/LConn1
  Simulink-PS Converter2/RConn1 -- OBang/LConn2
